simulink model "Simulink7"  (R2026a)
settings: Solver=ode45  StopTime=2  MaxStep=1e-4  RelTol=1e-6  AbsTol=1e-6

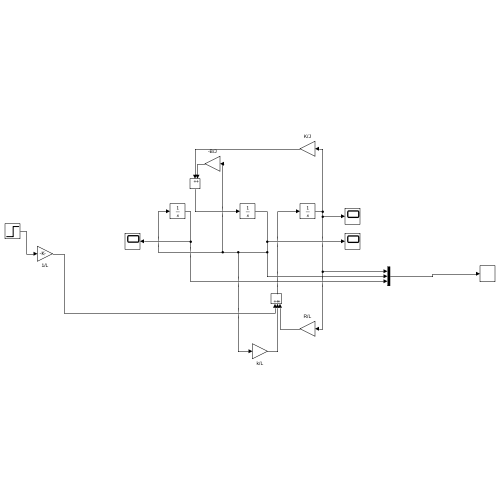
[thumbnail: Simulink's stored preview of the top-level diagram]
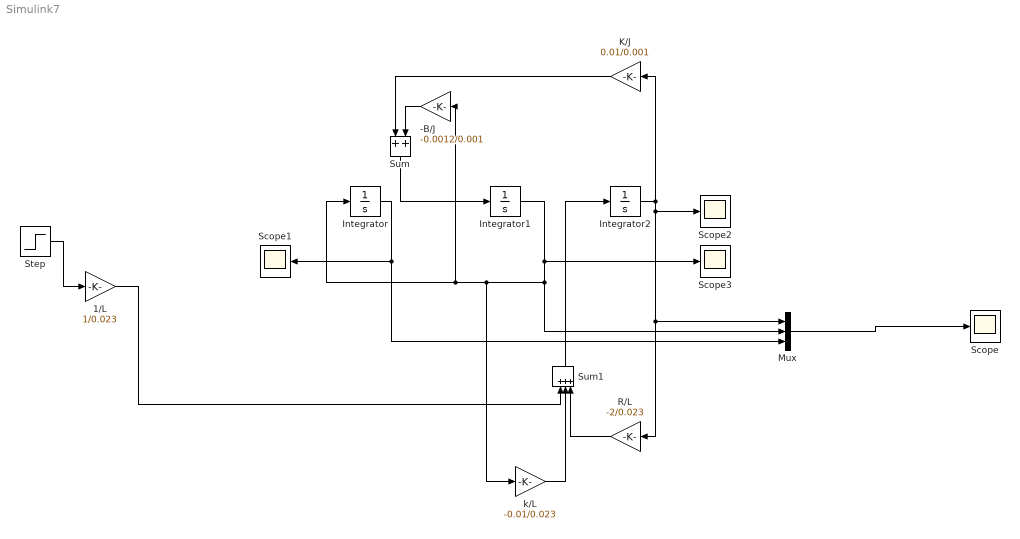
== system Simulink7 ==
  -B/J : Gain  Gain=-0.0012/0.001
  1/L : Gain  Gain=1/0.023
  Integrator : Integrator
  Integrator1 : Integrator
  Integrator2 : Integrator
  K/J : Gain  Gain=0.01/0.001
  Mux : Mux  Inputs=3
  R/L : Gain  Gain=-2/0.023
  Scope{,1..3} (4 alike) : Scope
      Scope settings: ActiveDisplayYMinimum=-7.5327054376238127  ActiveDisplayYMaximum=67.794348938614334
      Scope1 settings: ActiveDisplayYMinimum=-7.5327054376238127  ActiveDisplayYMaximum=67.794348938614334
      Scope2 settings: ActiveDisplayYMinimum=-0.74730749439094157  ActiveDisplayYMaximum=6.7257674495184752  DataLoggingVariableName=ScopeData2
      Scope3 settings: ActiveDisplayYMinimum=-5.5010271066051484  ActiveDisplayYMaximum=49.509243959446344  DataLoggingVariableName=ScopeData3
  Step : Step  Time=0  FinalValue=12  SampleTime=0
  Sum : Sum  Inputs=|++
  Sum1 : Sum  Inputs=|+++
  k/L : Gain  Gain=-0.01/0.023
  wires:
  Integrator1/1 -> Scope3/1, Mux/2, k/L/1, -B/J/1, Integrator/1
  Integrator2/1 -> Scope2/1, Mux/1, R/L/1, K/J/1
  Sum/1 -> Integrator1/1
  -B/J/1 -> Sum/2
  K/J/1 -> Sum/1
  Step/1 -> 1/L/1
  Sum1/1 -> Integrator2/1
  R/L/1 -> Sum1/3
  1/L/1 -> Sum1/1
  k/L/1 -> Sum1/2
  Mux/1 -> Scope/1
  Integrator/1 -> Scope1/1, Mux/3
